simulink model "main_model"  (R2025a)
settings: Solver=VariableStepAuto  StartTime=0.0  StopTime=1  RelTol=1e-3
libraries: spsGroundLib x2, eePwmGenerator x2, spsUniversalBridgeLib x2, spsSequenceAnalyzerLib x2, spsThreePhaseParallelRLCBranchLib x2, simulink_extras x1, spsSynchronousMachinepuStandardLib x1, spsThreePhasePISectionLineLib x1, spsThreePhaseParallelRLCLoadLib x1, spsThreePhaseSeriesRLCBranchLib x1, spsThreePhaseTransformerTwoWindingsLib x1, spsThreePhaseVIMeasurementLib x1
settings Model: Creator=smadh  LastModifiedBy=smadh
settings DataIOCC: SaveFormat=StructureWithTime  SaveOutput=off  SaveState=on  SignalLogging=off  DSMLogging=off  ReturnWorkspaceOutputs=off  LoggingToFile=on

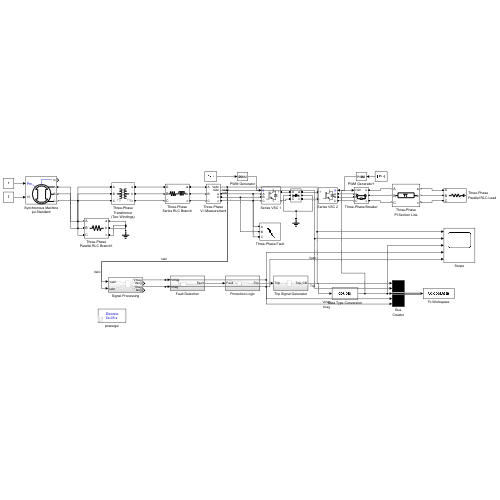
[thumbnail: Simulink's stored preview of the top-level diagram]
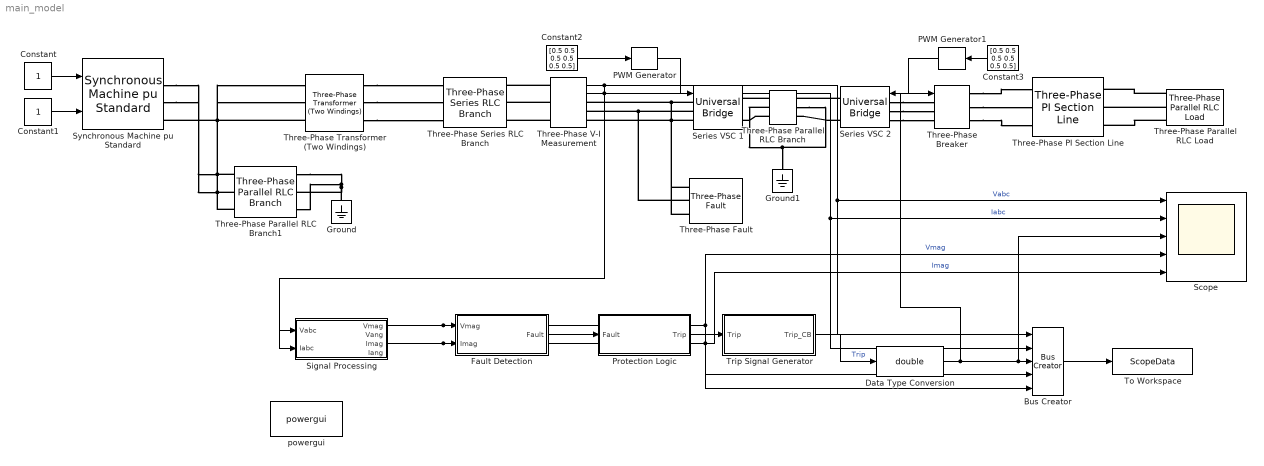
== system main_model ==
  Bus Creator : BusCreator  Inputs=5
  Constant : Constant
  Constant1 : Constant
  Constant2 : Constant  Value=[0.5 0.5 0.5 0.5 0.5 0.5]
  Constant3 : Constant  Value=[0.5 0.5 0.5 0.5 0.5 0.5]
  Data Type Conversion : DataTypeConversion  OutDataTypeStr=double  SaturateOnIntegerOverflow=off  RndMeth=Floor
  Fault Detection : Subsystem
  Ground : spsGroundLib/Ground  LConnTagsString=a
  Ground1 : spsGroundLib/Ground  LConnTagsString=a
  PWM Generator : eePwmGenerator/PWM Generator  CarrCount=Up  Tper=0.0005  Tdelay=0  Ts=5e-5
  PWM Generator1 : eePwmGenerator/PWM Generator  CarrCount=Up  Tper=0.0005  Tdelay=0  Ts=5e-5
  Protection Logic : Subsystem
  Scope : Scope  NumInputPorts=5
      settings: ShowGrid=off  ActiveDisplayYMinimum=-5799.0336252625048  ActiveDisplayYMaximum=6215.1524750098561
  Series VSC 1 : spsUniversalBridgeLib/Universal Bridge  Arms=3  SnubberResistance=1e5  SnubberCapacitance=inf  Device=IGBT / Diodes  Ron=1e-3  Lon=0  ForwardVoltages="[  0  0  ]"  ForwardVoltage=0  GTOparameters=[ 10e-6 , 20e-6 ]  IGBTparameters=[ 1e-6 , 2e-6 ]  Measurements=None  Measurements_2=None  converterType=Rectifier
  Series VSC 2 : spsUniversalBridgeLib/Universal Bridge  Arms=3  SnubberResistance=1e5  SnubberCapacitance=inf  Device=IGBT / Diodes  Ron=1e-3  Lon=0  ForwardVoltages="[  0  0  ]"  ForwardVoltage=0  GTOparameters=[ 10e-6 , 20e-6 ]  IGBTparameters=[ 1e-6 , 2e-6 ]  Measurements=None  Measurements_2=None  converterType=Rectifier
  Signal Processing : Subsystem
  Synchronous Machine pu Standard : spsSynchronousMachinepuStandardLib/Synchronous Machine pu Standard  PresetModel=No  MechanicalLoad=Mechanical power Pm  ShowDetailedParameters=on  RotorType=Salient-pole  Units=per unit standard parameters  MeasurementBus=off  NominalParameters=[10e6 11000 50]  Reactances1=[ 1.81, 0.3, 0.23, 1.76, 0.65, 0.25, 0.15 ]  Reactances2=[ 1.8 0.3 0.2 1.7 0.23 0.1 ]  dAxisTimeConstants=Short-circuit  qAxisTimeConstants=Short-circuit  TimeConstants1="[ 4.4849  0.0681  0.1  ]"  TimeConstants2=[ 8.0, 0.03, 1.0, 0.07 ]  TimeConstants3="[  4.49  0.0681  0.0513  ]"  TimeConstants4=[ 8.0, 0.03, 0.3371, 0.0295 ]  TimeConstants5=[ 1.01, 0.053, 0.1 ]  TimeConstants6=[ 1.3201, 0.023, 1.0, 0.07 ]  TimeConstants7=[0.012 0.003 0.003]  TimeConstants8=[ 1.3201, 0.0231, 0.3371, 0.0295 ]  StatorResistance=0.037875  Mechanical=[ 3.5 0 2 ]  PolePairs=20  InitialConditions=[0 0 1 1 1 0 -120 120 1]  SetSaturation=on  Saturation=[0.6404,0.7127,0.8441,0.9214,0.9956,1.082,1.19,1.316,1.457;0.7,0.7698,0.8872,0.9466,0.9969,1.046,1.1,1.151,1.201]  LoadFlowParameters=[1,0,0,0,0]  TsPowergui=0  TsBlock=-1  IterativeModel=Trapezoidal non iterative  IterativeDiscreteModel=Trapezoidal non iterative  BusType=swing  Pref=0  Qref=0  Qmin=-inf  Qmax=inf  PLF=0  QLF=0
  Three-Phase PI Section Line : spsThreePhasePISectionLineLib/Three-Phase PI Section Line  LConnTagsString=a|b|c  RConnTagsString=A|B|C  Length=100  Frequency=50  Resistances=[ 0.01273 0.3864]  Inductances="[ 0.9337e-3  4.1264e-3]"  Capacitances=[12.74e-9 7.751e-9]
  Three-Phase Parallel RLC Branch : spsThreePhaseParallelRLCBranchLib/Three-Phase Parallel RLC Branch  LConnTagsString=A|B|C  RConnTagsString=A|B|C  BranchType=C  Resistance=1  Inductance=1e-3  Capacitance=1e-6  Measurements=None
  Three-Phase Parallel RLC Branch1 : spsThreePhaseParallelRLCBranchLib/Three-Phase Parallel RLC Branch  LConnTagsString=A|B|C  RConnTagsString=A|B|C  BranchType=R  Resistance=10  Inductance=Inf  Capacitance=0  Measurements=None
  Three-Phase Parallel RLC Load : spsThreePhaseParallelRLCLoadLib/Three-Phase Parallel RLC Load  LConnTagsString=A|B|C  Configuration=Y (grounded)  NominalVoltage=11000  Vabc=[1e3 1e3 1e3]  Vabcp=[1e3 1e3 1e3]  NominalFrequency=50  UnbalancedPower=off  ActivePower=500e6  InductivePower=0  CapacitivePower=0  Pabc=[10e3 9e3 11e3]  QLabc=[100 90 110]  QCabc=[100 90 110]  Pabcp=[10e3 9e3 11e3]  QLabcp=[100 90 110]  QCabcp=[100 90 110]  Measurements=None  LoadType=constant Z
  Three-Phase Series RLC Branch : spsThreePhaseSeriesRLCBranchLib/Three-Phase Series RLC Branch  LConnTagsString=A|B|C  RConnTagsString=A|B|C  BranchType=RL  Resistance=0.001  Inductance=1e-3  Capacitance=1e-6  Measurements=None
  Three-Phase Transformer (Two Windings) : spsThreePhaseTransformerTwoWindingsLib/Three-Phase Transformer (Two Windings)  Winding1Connection=Yg  Winding2Connection=Yg  CoreType=Three single-phase transformers  SetSaturation=off  Hysteresis=off  DataFile='hysteresis'  SetInitialFlux=off  Measurements=None  UNITS=pu  NominalPower=[ 5e6 , 50 ]  Winding1=[ 11000 , 0.002 , 0.08 ]  Winding2=[ 415 , 0.002 , 0.08 ]  Rm=500  Lm=500  L0=0.5  Saturation=[ 0,0 ; 0.0024,1.2 ; 1.0,1.52 ]  InitialFluxes=[ 0.8 , -0.8 , 0.7 ]  BreakLoop=off  DiscreteSolver=Trapezoidal iterative  DataType=off  TransfoNumber=1
  Three-Phase V-I Measurement : spsThreePhaseVIMeasurementLib/Three-Phase V-I Measurement  VoltageMeasurement=phase-to-phase  SetLabelV=off  LabelV=Vabc  Vpu=off  VpuLL=off  CurrentMeasurement=yes  SetLabelI=off  LabelI=Iabc  Ipu=off  Pbase=100e6  Vbase=500e3  OutputType=Complex  PhasorSimulation=off  PSBequivalent=0
  Three-Phase Breaker : spsThreePhaseBreakerLib/Three-Phase Breaker  InitialState=closed  SwitchA=on  SwitchB=on  SwitchC=on  SwitchTimes="[0.2  0.4]"  External=on  BreakerResistance=0.001  SnubberResistance=1e6  SnubberCapacitance=inf  Measurements=None
  Three-Phase Fault : spsThreePhaseFaultLib/Three-Phase Fault  InitialStates=0  FaultA=on  FaultB=on  FaultC=on  GroundFault=on  SwitchTimes="[0.2  0.4]"  External=off  SwitchStatus=NaN  FaultResistance=0.001  GroundResistance=0.01  SnubberResistance=1e6  SnubberCapacitance=inf  Measurements=None
  To Workspace : ToWorkspace  VariableName=ScopeData  SaveFormat=Structure With Time  SampleTime=-1
  Trip Signal Generator : Subsystem
  powergui : spspowerguiLib/powergui  Priority=1  SimulationMode=Discrete  SampleTime=5e-5  frequency=60  Iterations=50  frequencyindice=50  Pbase=100e6  ErrMax=1e-4  UnitsV=kV  UnitsW=MW  buscounter=0  FunctionMessages=off  echomessages=off  EnableUseOfTLC=off  CurrentSourceSwitches=off  DisableSnubberDevices=off  DisableRonSwitches=off  DisableVfSwitches=off  DisplayEquations=off  AutomaticDiscreteSolvers=on  SolverType=Tustin/Backward Euler (TBE)  Interpol=off  ExternalGateDelay=off  methode=off  Ts=100  x0status=blocks  SPID=on  SwTol=0  HookPort=off  NonlinearTolerance=1e-4  nMaxIteration=100  ContinueOnMaxIteration=off  RestoreLinks=warning  ResistiveCurrentMeasurement=off  Frange=[0:2:500]  Ylog=off  Xlog=on  ShowGrid=off  save=off  variable=ZData  structure=0  ZoomFFT=off  StartTime=0.0  cycles=1  DisplayStyle=1  fundamental=60  FreqAxis=off  MaxFrequency=1000  frequencyindicesteady=1  RmsSteady=1  display=off
  wires:
  Three-Phase V-I Measurement/1 -> Bus Creator/1, Scope/1, Signal Processing/1(Vabc)  "Vabc"
  Three-Phase V-I Measurement/2 -> Bus Creator/2, Scope/2, Signal Processing/2(Iabc)  "Iabc"
  Fault Detection/1(Fault) -> Protection Logic/1(Fault)
  Protection Logic/1(Trip) -> Trip Signal Generator/1(Trip)
  Data Type Conversion/1 -> Bus Creator/3, Scope/3, Three-Phase Breaker/1
  Bus Creator/1 -> To Workspace/1
  Signal Processing/3(Imag) -> Bus Creator/5, Scope/5, Fault Detection/2(Imag)  "Imag"
  Signal Processing/1(Vmag) -> Bus Creator/4, Scope/4, Fault Detection/1(Vmag)  "Vmag"
  Constant/1 -> Synchronous Machine pu Standard/1
  Constant1/1 -> Synchronous Machine pu Standard/2
  Trip Signal Generator/1(Trip_CB) -> Data Type Conversion/1  "Trip"
  PWM Generator/1 -> Series VSC 1/1
  Constant2/1 -> PWM Generator/1
  PWM Generator1/1 -> Series VSC 2/1
  Constant3/1 -> PWM Generator1/1
  connections:
  Three-Phase Transformer (Two Windings)/RConn1 -- Three-Phase Series RLC Branch/LConn1
  Three-Phase Transformer (Two Windings)/RConn2 -- Three-Phase Series RLC Branch/LConn2
  Three-Phase Transformer (Two Windings)/RConn3 -- Three-Phase Series RLC Branch/LConn3
  Three-Phase Breaker/RConn1 -- Three-Phase PI Section Line/LConn1
  Three-Phase Breaker/RConn2 -- Three-Phase PI Section Line/LConn2
  Three-Phase Breaker/RConn3 -- Three-Phase PI Section Line/LConn3
  Three-Phase Parallel RLC Load/LConn2 -- Three-Phase PI Section Line/RConn2
  Three-Phase Parallel RLC Load/LConn1 -- Three-Phase PI Section Line/RConn1
  Three-Phase Parallel RLC Load/LConn3 -- Three-Phase PI Section Line/RConn3
  Synchronous Machine pu Standard/RConn1 -- Three-Phase Parallel RLC Branch1/LConn1 -- Three-Phase Transformer (Two Windings)/LConn1
  Synchronous Machine pu Standard/RConn2 -- Three-Phase Parallel RLC Branch1/LConn2 -- Three-Phase Transformer (Two Windings)/LConn2
  Three-Phase Transformer (Two Windings)/LConn3 -- Three-Phase Parallel RLC Branch1/LConn3 -- Synchronous Machine pu Standard/RConn3
  Three-Phase Parallel RLC Branch1/RConn1 -- Ground/LConn1 -- Three-Phase Parallel RLC Branch1/RConn2 -- Three-Phase Parallel RLC Branch1/RConn3
  Three-Phase V-I Measurement/LConn2 -- Three-Phase Series RLC Branch/RConn2
  Three-Phase V-I Measurement/LConn1 -- Three-Phase Series RLC Branch/RConn1
  Three-Phase V-I Measurement/LConn3 -- Three-Phase Series RLC Branch/RConn3
  Three-Phase Fault/LConn3 -- Three-Phase V-I Measurement/RConn3 -- Series VSC 1/LConn3
  Three-Phase Fault/LConn2 -- Three-Phase V-I Measurement/RConn2 -- Series VSC 1/LConn2
  Three-Phase Fault/LConn1 -- Three-Phase V-I Measurement/RConn1 -- Series VSC 1/LConn1
  Three-Phase Parallel RLC Branch/LConn1 -- Series VSC 1/RConn1
  Three-Phase Parallel RLC Branch/LConn3 -- Series VSC 1/RConn2
  Series VSC 2/LConn1 -- Three-Phase Breaker/LConn1
  Series VSC 2/LConn2 -- Three-Phase Breaker/LConn2
  Series VSC 2/LConn3 -- Three-Phase Breaker/LConn3
  Series VSC 2/RConn2 -- Three-Phase Parallel RLC Branch/RConn3
  Series VSC 2/RConn1 -- Three-Phase Parallel RLC Branch/RConn1
  Three-Phase Parallel RLC Branch/RConn2 -- Three-Phase Parallel RLC Branch/LConn2 -- Ground1/LConn1

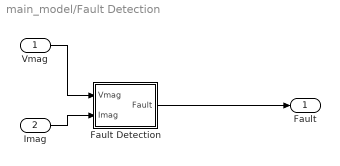
== system main_model/Fault Detection ==
  Vmag : Inport
  Imag : Inport  Port=2
  Fault Detection : Subsystem
  Fault : Outport
  wires:
  Vmag/1 -> Fault Detection/1(Vmag)
  Imag/1 -> Fault Detection/2(Imag)
  Fault Detection/1(Fault) -> Fault/1

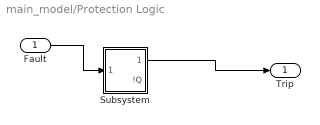
== system main_model/Protection Logic ==
  Fault : Inport
  Subsystem : Subsystem
  Trip : Outport
  wires:
  Fault/1 -> Subsystem/1(Fault)
  Subsystem/1(Trip) -> Trip/1

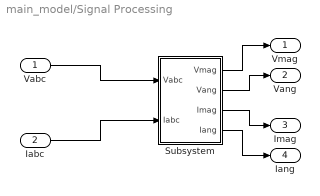
== system main_model/Signal Processing ==
  Vabc : Inport
  Iabc : Inport  Port=2
  Subsystem : Subsystem
  Vmag : Outport
  Vang : Outport  Port=2
  Imag : Outport  Port=3
  Iang : Outport  Port=4
  wires:
  Vabc/1 -> Subsystem/1(Vabc)
  Iabc/1 -> Subsystem/2(Iabc)
  Subsystem/1(Vmag) -> Vmag/1
  Subsystem/2(Vang) -> Vang/1
  Subsystem/3(Imag) -> Imag/1
  Subsystem/4(Iang) -> Iang/1

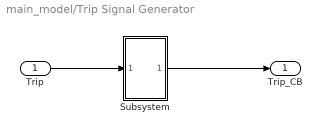
== system main_model/Trip Signal Generator ==
  Trip : Inport
  Subsystem : Subsystem
  Trip_CB : Outport
  wires:
  Trip/1 -> Subsystem/1(Trip)
  Subsystem/1(Trip_CB) -> Trip_CB/1

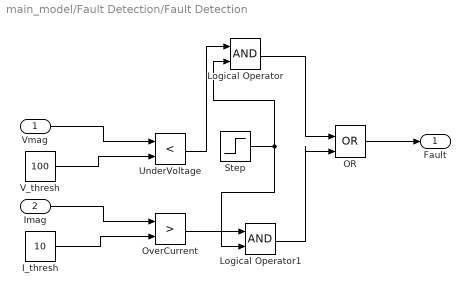
== system main_model/Fault Detection/Fault Detection ==
  Vmag : Inport
  Imag : Inport  Port=2
  I_thresh : Constant  Value=10
  Logical Operator : Logic  AllPortsSameDT=off  OutDataTypeStr=boolean
  Logical Operator1 : Logic  AllPortsSameDT=off  OutDataTypeStr=boolean
  OR : Logic  Operator=OR  IconShape=distinctive  AllPortsSameDT=off  OutDataTypeStr=boolean
  OverCurrent : RelationalOperator  Operator=>  OutDataTypeStr=boolean  RndMeth=Simplest  InputSameDT=off
  Step : Step  Time=0.15  SampleTime=0
  UnderVoltage : RelationalOperator  Operator=<  OutDataTypeStr=boolean  RndMeth=Simplest  InputSameDT=off
  V_thresh : Constant  Value=100
  Fault : Outport
  wires:
  Vmag/1 -> UnderVoltage/1
  V_thresh/1 -> UnderVoltage/2
  Imag/1 -> OverCurrent/1
  I_thresh/1 -> OverCurrent/2
  OR/1 -> Fault/1
  UnderVoltage/1 -> Logical Operator/1
  Step/1 -> Logical Operator1/2, Logical Operator/2
  Logical Operator/1 -> OR/1
  OverCurrent/1 -> Logical Operator1/1
  Logical Operator1/1 -> OR/2

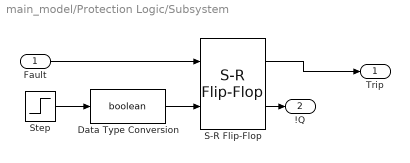
== system main_model/Protection Logic/Subsystem ==
  Fault : Inport
  Data Type Conversion : DataTypeConversion  OutDataTypeStr=boolean  SaturateOnIntegerOverflow=off  RndMeth=Floor
  S-R Flip-Flop : simulink_extras/Flip Flops/S-R Flip-Flop  initial_condition=0
  Step : Step  Time=0.4  SampleTime=0
  Trip : Outport
  !Q : Outport  Port=2
  wires:
  S-R Flip-Flop/1 -> Trip/1
  S-R Flip-Flop/2 -> !Q/1
  Data Type Conversion/1 -> S-R Flip-Flop/2
  Step/1 -> Data Type Conversion/1
  Fault/1 -> S-R Flip-Flop/1

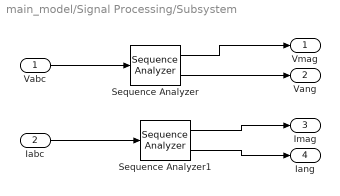
== system main_model/Signal Processing/Subsystem ==
  Vabc : Inport
  Iabc : Inport  Port=2
  Sequence Analyzer : spsSequenceAnalyzerLib/Sequence Analyzer  Freq=50  n=1  seq=Positive  InInit=[140, 0]  Ts=5e-5
      settings: LibrarySourceBlock=sps_lib/Sensors and Measurements/Sequence Analyzer
  Sequence Analyzer1 : spsSequenceAnalyzerLib/Sequence Analyzer  Freq=50  n=1  seq=Positive  InInit=[1, 0]  Ts=5e-5
      settings: LibrarySourceBlock=sps_lib/Sensors and Measurements/Sequence Analyzer
  Vmag : Outport
  Vang : Outport  Port=2
  Imag : Outport  Port=3
  Iang : Outport  Port=4
  wires:
  Iabc/1 -> Sequence Analyzer1/1
  Sequence Analyzer1/2 -> Iang/1
  Vabc/1 -> Sequence Analyzer/1
  Sequence Analyzer/2 -> Vang/1
  Sequence Analyzer1/1 -> Imag/1
  Sequence Analyzer/1 -> Vmag/1

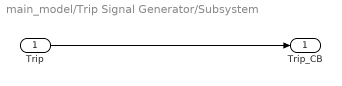
== system main_model/Trip Signal Generator/Subsystem ==
  Trip : Inport
  Trip_CB : Outport
  wires:
  Trip/1 -> Trip_CB/1
